simulink model "modelo_3_naolinear"  (R2026a)
settings: Solver=ode45  StopTime=8
libraries: cstblocks_lti x2

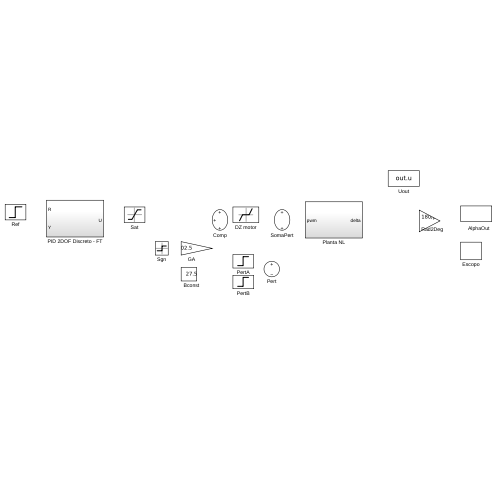
[thumbnail: Simulink's stored preview of the top-level diagram]
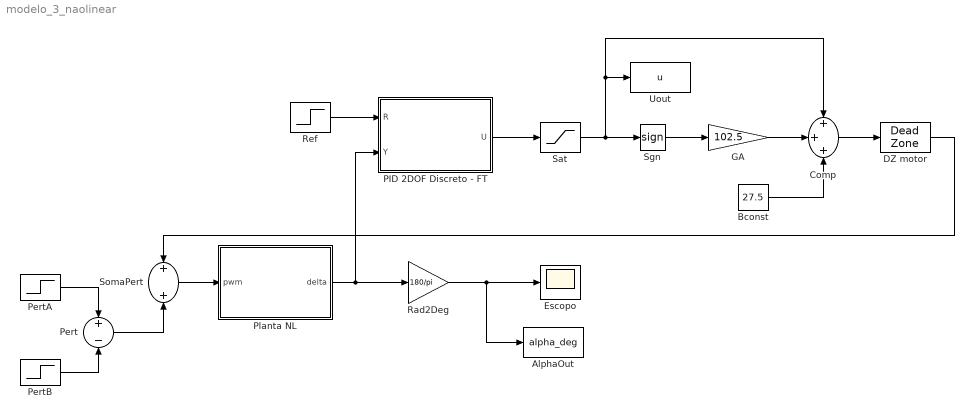
== system modelo_3_naolinear ==
  AlphaOut : ToWorkspace  VariableName=alpha_deg  SaveFormat=Timeseries  SampleTime=-1
  Bconst : Constant  Value=27.5
  Comp : Sum  Inputs=+++
  DZ motor : DeadZone  LowerValue=-75  UpperValue=130
  Escopo : Scope
  GA : Gain  Gain=102.5
  PID 2DOF Discreto - FT : Subsystem
  Pert : Sum  Inputs=+-
  PertA : Step  Time=2  FinalValue=60  SampleTime=0
  PertB : Step  Time=2.3  FinalValue=60  SampleTime=0
  Planta NL : Subsystem
  Rad2Deg : Gain  Gain=180/pi
  Ref : Step  Time=0  FinalValue=0  SampleTime=0
  Sat : Saturate  UpperLimit=255  LowerLimit=-255
  Sgn : Signum
  SomaPert : Sum
  Uout : ToWorkspace  VariableName=u  SaveFormat=Timeseries  SampleTime=-1
  wires:
  DZ motor/1 -> SomaPert/1
  Pert/1 -> SomaPert/2
  PertB/1 -> Pert/2
  Sat/1 -> Uout/1, Comp/1, Sgn/1
  GA/1 -> Comp/2
  Ref/1 -> PID 2DOF Discreto - FT/1(R)
  SomaPert/1 -> Planta NL/1(pwm)
  Planta NL/1(delta) -> PID 2DOF Discreto - FT/2(Y), Rad2Deg/1
  Bconst/1 -> Comp/3
  PertA/1 -> Pert/1
  PID 2DOF Discreto - FT/1(U) -> Sat/1
  Sgn/1 -> GA/1
  Rad2Deg/1 -> Escopo/1, AlphaOut/1
  Comp/1 -> DZ motor/1

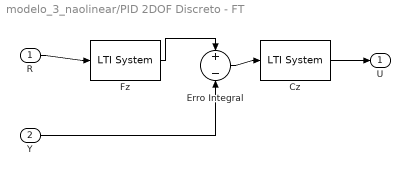
== system modelo_3_naolinear/PID 2DOF Discreto - FT ==
  R : Inport
  Y : Inport  Port=2
  Cz : cstblocks_lti/LTI System  sys=Cz  IC=[]  PadeOrder=0
      settings: LibrarySourceBlock=cstblocks/LTI System
  Erro Integral : Sum  Inputs=+-
  Fz : cstblocks_lti/LTI System  sys=Fz  IC=[]  PadeOrder=0
      settings: LibrarySourceBlock=cstblocks/LTI System
  U : Outport
  wires:
  R/1 -> Fz/1
  Fz/1 -> Erro Integral/1
  Y/1 -> Erro Integral/2
  Erro Integral/1 -> Cz/1
  Cz/1 -> U/1

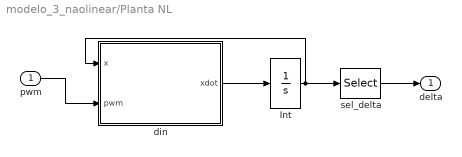
== system modelo_3_naolinear/Planta NL ==
  pwm : Inport
  Int : Integrator  InitialCondition=[0;0;0;0]
  din : MATLAB Function  TreatAsAtomicUnit=on
  sel_delta : Selector  InputPortWidth=4  IndexOptions=Index vector (dialog)  Indices=2  OutputSizes=1
  delta : Outport
  wires:
  pwm/1 -> din/2(pwm)
  Int/1 -> din/1(x), sel_delta/1
  din/1(xdot) -> Int/1
  sel_delta/1 -> delta/1

== matlab function modelo_3_naolinear/Planta NL/din ==
  data: x input; xdot output; pwm input
function xdot = din(x, pwm)
%#codegen
k_tau = 0.00050868; Ib = 0.0015; mp = 0.045; Lb = 0.12; J = 0.00051271;
lp = 0.08; b_th = 1e-05; b_al = 0.00057586; g = 9.81;
th_d = x(3); d = x(2); d_d = x(4);
tau  = k_tau*pwm;
M11 = Ib + mp*Lb^2 + J*sin(d)^2;
M12 = -mp*Lb*lp*cos(d);
M22 = J;
C1  = J*sin(2*d)*th_d*d_d + mp*Lb*lp*sin(d)*d_d^2;
C2  = -0.5*J*sin(2*d)*th_d^2;
r1  = tau - C1 - b_th*th_d;
r2  =     - C2 - b_al*d_d - mp*g*lp*sin(d);
det = M11*M22 - M12^2;
th_dd = ( M22*r1 - M12*r2)/det;
d_dd  = (-M12*r1 + M11*r2)/det;
xdot  = [th_d; d_d; th_dd; d_dd];
